simulink model "EINT_RL_closed_loop_xy"  (R2025b)
settings: Solver=FixedStepAuto  StartTime=0.0  StopTime=T_end  FixedStep=Ts  RelTol=1e-3
values from neighbouring files (symbols this model uses):
  Ts = 0.05    [EINT_RL_eval_xy.m]
undefined symbols (not defined in the file or in its folder): rl_controller_xy
settings Model: Creator=anoua  LastModifiedBy=anoua

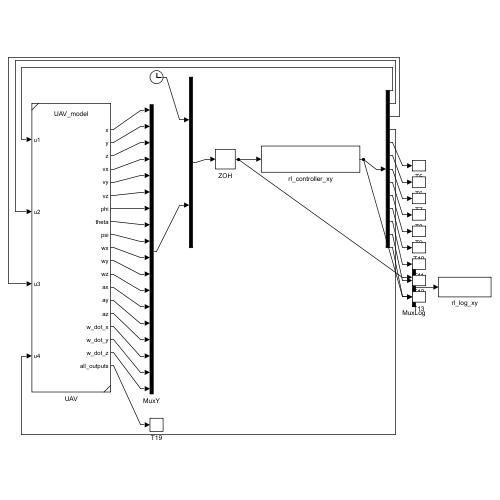
[thumbnail: Simulink's stored preview of the top-level diagram]
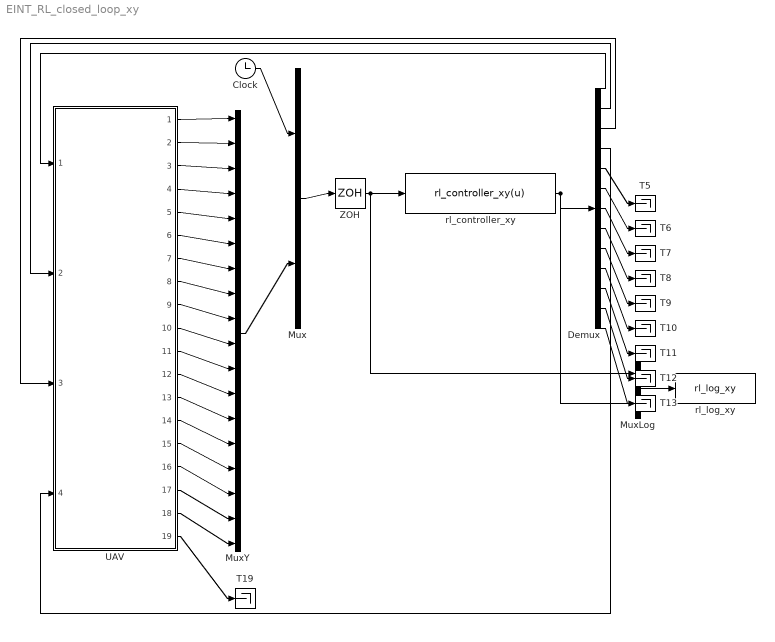
== system EINT_RL_closed_loop_xy ==
  Clock : Clock
  Demux : Demux  Outputs=13
  Mux : Mux  Inputs=2
  MuxLog : Mux  Inputs=2
  MuxY : Mux  Inputs=18
  T{5..13,19} (10 alike) : Terminator
  UAV : Subsystem  ReferencedSubsystem=UAV_model
  ZOH : ZeroOrderHold  SampleTime=Ts
  rl_controller_xy : MATLABFcn  MATLABFcn=rl_controller_xy(u)  OutputDimensions=13  SampleTime=Ts
  rl_log_xy : ToWorkspace  VariableName=rl_log_xy  SampleTime=Ts
  wires:
  UAV/19 -> T19/1
  UAV/1 -> MuxY/1
  UAV/2 -> MuxY/2
  UAV/3 -> MuxY/3
  UAV/4 -> MuxY/4
  UAV/5 -> MuxY/5
  UAV/6 -> MuxY/6
  UAV/7 -> MuxY/7
  UAV/8 -> MuxY/8
  UAV/9 -> MuxY/9
  UAV/10 -> MuxY/10
  UAV/11 -> MuxY/11
  UAV/12 -> MuxY/12
  UAV/13 -> MuxY/13
  UAV/14 -> MuxY/14
  UAV/15 -> MuxY/15
  UAV/16 -> MuxY/16
  UAV/17 -> MuxY/17
  UAV/18 -> MuxY/18
  Clock/1 -> Mux/1
  MuxY/1 -> Mux/2
  Mux/1 -> ZOH/1
  ZOH/1 -> rl_controller_xy/1, MuxLog/1
  rl_controller_xy/1 -> Demux/1, MuxLog/2
  Demux/1 -> UAV/1
  Demux/2 -> UAV/2
  Demux/3 -> UAV/3
  Demux/4 -> UAV/4
  Demux/5 -> T5/1
  Demux/6 -> T6/1
  Demux/7 -> T7/1
  Demux/8 -> T8/1
  Demux/9 -> T9/1
  Demux/10 -> T10/1
  Demux/11 -> T11/1
  Demux/12 -> T12/1
  Demux/13 -> T13/1
  MuxLog/1 -> rl_log_xy/1
